simulink model "SYS_CL_Z_ref"  (R2026a)
settings: Solver=VariableStepAuto  StopTime=150.0
undefined symbols (not defined in the file): K_d_z_ref, K_p_z_ref
libraries: cstblocks_lti x1
settings Model: Creator=samuel  LastModifiedBy=samuel

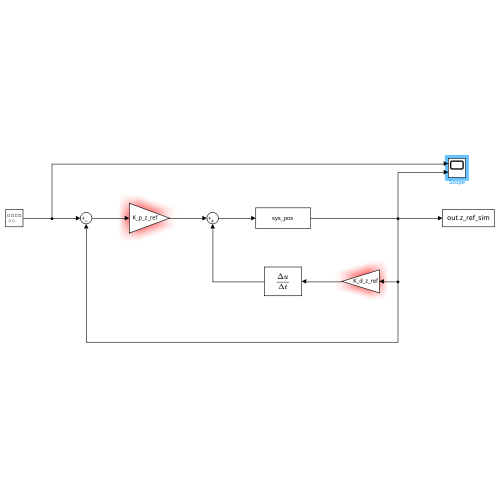
[thumbnail: Simulink's stored preview of the top-level diagram]
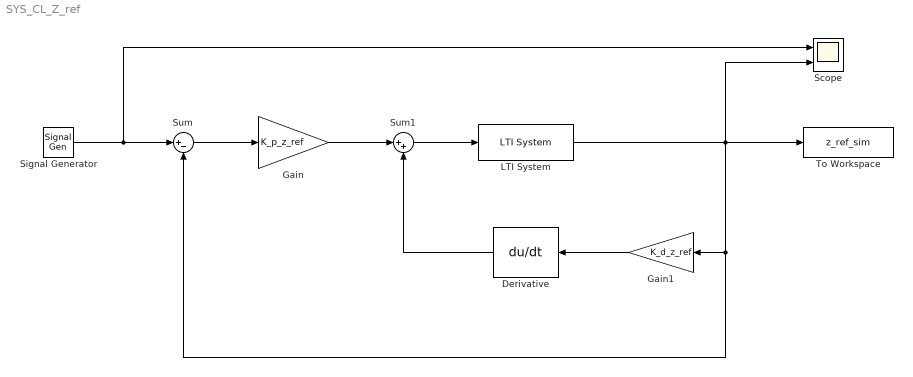
== system SYS_CL_Z_ref ==
  Derivative : Derivative
  Gain : Gain  Gain=K_p_z_ref
  Gain1 : Gain  Gain=K_d_z_ref
  LTI System : cstblocks_lti/LTI System  sys=sys_pos  IC=[]  PadeOrder=0
      settings: LibrarySourceBlock=cstblocks/LTI System
  Scope : Scope  NumInputPorts=2
      settings: ActiveDisplayYMinimum=-46.521904564763332  ActiveDisplayYMaximum=66.940240296216245
  Signal Generator : SignalGenerator  WaveForm=square  Amplitude=30  Frequency=0.01
  Sum : Sum  Inputs=|+-
  Sum1 : Sum  Inputs=|++
  To Workspace : ToWorkspace  VariableName=z_ref_sim  SaveFormat=Timeseries  SampleTime=-1
  wires:
  Sum/1 -> Gain/1
  Signal Generator/1 -> Scope/1, Sum/1
  Sum1/1 -> LTI System/1
  Gain/1 -> Sum1/1
  Gain1/1 -> Derivative/1
  Derivative/1 -> Sum1/2
  LTI System/1 -> Scope/2, To Workspace/1, Gain1/1, Sum/2
